simulink model "battery"  (R2024a)
settings: Solver=ode23t  StartTime=0.0  StopTime=10000.0  MaxStep=5e-2  RelTol=1e-3
undefined symbols (not defined in the file or in its folder): battery_builder_rtmsupport, gcbh
libraries: fl_lib x8, batt_lib x8, nesl_utility x6, Batteries_thermal_lib x6, SimscapeFluids_lib x1, simulink x1
(part 1 of 2)
settings Model: Creator=amtha  LastModifiedBy=amtha

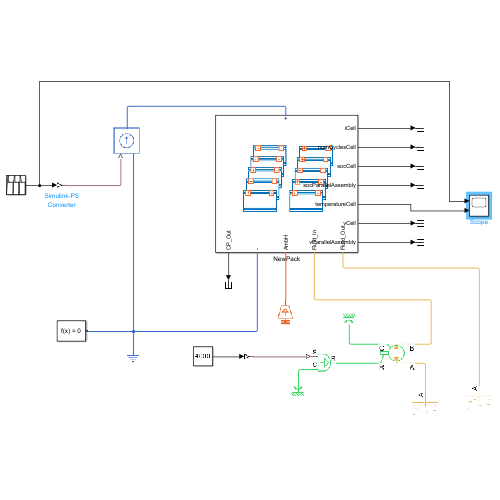
[thumbnail: Simulink's stored preview of the top-level diagram]
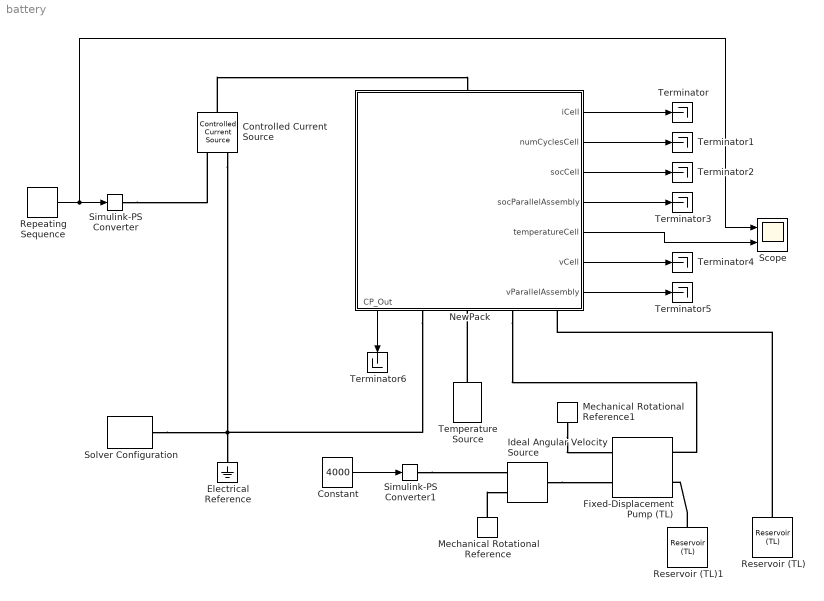
== system battery ==
  Constant : Constant  Value=4000
  Controlled Current Source : fl_lib/Electrical/Electrical Sources/Controlled Current Source
  Electrical Reference : fl_lib/Electrical/Electrical Elements/Electrical Reference
  Fixed-Displacement Pump (TL) : SimscapeFluids_lib/Thermal Liquid/Pumps & Motors/Fixed-Displacement Pump (TL)  loss_spec=fluids.thermal_liquid.pumps_motors.enum.LossSpec.Analytical  displacement=30 cm^3/rev  omega_nominal=4000 rpm  p_nominal=10 MPa  mu_nominal=0.9 cP  vol_eff_nominal=0.92  mech_eff_nominal=0.88  no_load_torque=0 N*m  p_diff_eff_TLU=[.1, 1, 2] MPa  omega_eff_TLU=[250, 500, 1000, 2000, 3000, 4000] rpm  vol_eff_TLU=[.816, .908, .954, .977, .981, .984; .325, .663, .831, .916, .925, .946; .137, .568, .78, .892, .893, .91]  mech_eff_TLU=[.996, .996, .996, .996, .996, .996; .988, .989, .989, .989, .989, .99; .981, .981, .982, .982, .983, .984]  p_diff_loss_TLU=[.1, 1, 2] MPa  omega_loss_TLU=[250, 500, 1000, 2000, 3000, 4000] rpm  vol_loss_TLU=1e-3 * [.023, .023, .023, .023, .0285, .032; .0844, .0842, .0845, .084, .1125, .108; .1079, .108, .11, .108, .1605, .18] m^3/s  mech_loss_TLU=[.002, .002, .002, .002, .002, .002; .0607, .0556, .0556, .0556, .0556, .0505; .1937, .1937, .1833, .1833, .1729, .1626] N*m  vol_eff_min=1e-3  vol_eff_max=1  mech_eff_min=1e-3  mech_eff_max=1  pressure_threshold=1e-3 MPa  omega_threshold=100 rpm  area=4.9087 cm^2  supplied_range_check=simscape.enum.assert.action.none  pump_mode_check=simscape.enum.assert.action.none
  Ideal Angular Velocity Source : fl_lib/Mechanical/Mechanical Sources/Ideal Angular Velocity Source
  Mechanical Rotational Reference : fl_lib/Mechanical/Rotational Elements/Mechanical Rotational Reference
  Mechanical Rotational Reference1 : fl_lib/Mechanical/Rotational Elements/Mechanical Rotational Reference
  NewPack : Subsystem  LoadFcn=battery_builder_rtmsupport('loadfcn',gcbh);
      settings: CopyFcn=battery_builder_rtmsupport('copyfcn',gcbh);  PreCopyFcn=battery_builder_rtmsupport('precopyfcn',gcbh);  PreDeleteFcn=battery_builder_rtmsupport('predeletefcn',gcbh);  PortSchema="{\"entries\":[{\"content\":{\"sides\":[{\"content\":{\"connectorIds\":[\"LConn1\"]},\"type\":\"ConnectorPlacement.EquallySpacedRectSide\",\"uuid\":\"1e77f675-d87b-42aa-aa84-96264be7bb8b\"},{\"content\":{\"connectorIds\":[\"Out1\",\"RConn1\",\"RConn2\",\"RConn3\",\"RConn4\"],\"side\":\"RIGHT\"},\"type\":\"ConnectorPlacement.EquallySpacedRectSide\",\"uuid\":\"6d3cd395-a28c-44d8-a256-e39544efc771\"},{\"content\":{\"side\":\"TOP\"},\"type\":\"ConnectorPlacement.EquallySpacedRectSide\",\"uuid\":\"362665c8-a493-42c4-a520-da428b1848bf\"},{\"content\":{\"connectorIds\":[\"Out2\",\"Out3\",\"Out4\",\"Out5\",\"Out6\",\"Out7\",\"Out8\"],\"side\":\"BOTTOM\"},\"type\":\"ConnectorPlacement.EquallySpacedRectSide\",\"uuid\":\"f34d4770-2d50-43cb-948c-fae9218760e2\"}]},\"type\":\"ConnectorPlacement.EquallySpacedConnector\",\"uuid\":\"a7a1b69c-e4ee-453d-b7ec-7a49ac1cf5a9\"}],\"packageUris\":[\"http://schema.mathworks.com/mf0/Connector/R2020b\"],\"version\":\"1.0\"}"
      mask Display: image('$imagefile')
  Repeating Sequence : simulink/Sources/Repeating Sequence  rep_seq_t=[0 500 1000 1500 2000 3000 3500 4000 5000 10000]  rep_seq_y=[-10 -10 0 0 5 5 0 0 0 0]
  Reservoir (TL) : fl_lib/Thermal Liquid/Elements/Reservoir (TL)  pressure_spec=foundation.enum.pressure_spec.atmospheric  reservoir_pressure=0.101325 MPa  reservoir_temperature=293.15 K  area=0.01 m^2
  Reservoir (TL)1 : fl_lib/Thermal Liquid/Elements/Reservoir (TL)  pressure_spec=foundation.enum.pressure_spec.atmospheric  reservoir_pressure=0.101325 MPa  reservoir_temperature=30 degC  area=0.01 m^2
  Scope : Scope  NumInputPorts=2
  Simulink-PS Converter : nesl_utility/Simulink-PS Converter  PhysicalDomain=network_engine_domain  SubClassName=ps_input  LeftPortType=input  RightPortType=output  PseudoPeriodic=off  Frequencies=[]  NoiseDistribution=none  NoiseParameters=[]  Unit=1  AffineConversion=off  FilteringAndDerivatives=provide  SimscapeFilterOrder=1  InputFilterTimeConstant=0.001  UdotUserProvided=0
  Simulink-PS Converter1 : nesl_utility/Simulink-PS Converter  PhysicalDomain=network_engine_domain  SubClassName=ps_input  LeftPortType=input  RightPortType=output  PseudoPeriodic=off  Frequencies=[]  NoiseDistribution=none  NoiseParameters=[]  Unit=1  AffineConversion=off  FilteringAndDerivatives=provide  SimscapeFilterOrder=1  InputFilterTimeConstant=0.001  UdotUserProvided=0
  Solver Configuration : nesl_utility/Solver Configuration  PhysicalDomain=network_engine_domain  SubClassName=solver  LeftPortType=input  RightPortType=generic  Tones=[]  Harmonics=[]  SimulateNoise=off  Profile=off  UseLocalSampling=off  EnableSwitchedLinearOptims=on  FrequencyDomain=off  UseCCode=off  RelTol=0.001  AbsTol=0.001  MinStep=1e-09  ToWorkspace=off  RevertToSquareIcSolve=off  NumHomotopyIterations=100  PhasorMode=off  PhasorModeNumHarmonics=1  ConsistencySolver=NEWTON_XTOL_AFTER_FTOL  IndexReductionMethod=DerivativeReplacement  DoDC=off  ResidualTolerance=1e-09  ConsistencyTolSource=GLOBAL  ConsistencyAbsTol=0.001  ConsistencyRelTol=0.001  ConsistencyTolFactor=0.001  UseLocalSolver=off  LocalSolverChoice=NE_BACKWARD_EULER_ADVANCER  ResolveIndetEquations=on  FunctionEvalNumThread=1  LocalSolverSampleTime=0.001  DoFixedCost=off  MaxNonlinIter=3  MaxModeIter=2  ComputeImpulses=off  ImpulseIterations=2  LinearAlgebra=auto  LinearAlgebraNumThread=0  EquationFormulation=NE_TIME_EF  DelaysMemoryBudget=1024  AutomaticFiltering=on  FilteringTimeConstant=0.001  PartitionStorageMethod=AS_NEEDED  PartitionMemoryBudget=1024  PartitionMethod=ROBUST  MultibodyUseLocalSolver=off  MultibodyLocalSolverChoice=ODE1  MultibodyLocalSolverSampleTime=0.001
  Temperature Source : fl_lib/Thermal/Thermal Sources/Temperature Source  temperature=293.15 K
  Terminator{,1..6} (7 alike) : Terminator
  wires:
  NewPack/2(iCell) -> Terminator/1
  NewPack/3(numCyclesCell) -> Terminator1/1
  NewPack/4(socCell) -> Terminator2/1
  NewPack/5(socParallelAssembly) -> Terminator3/1
  NewPack/7(vCell) -> Terminator4/1
  NewPack/8(vParallelAssembly) -> Terminator5/1
  NewPack/1(CP_Out) -> Terminator6/1
  Repeating Sequence/1 -> Scope/1, Simulink-PS Converter/1
  NewPack/6(temperatureCell) -> Scope/2
  Constant/1 -> Simulink-PS Converter1/1
  connections:
  Simulink-PS Converter/RConn1 -- Controlled Current Source/RConn1
  Controlled Current Source/RConn2 -- Solver Configuration/RConn1 -- NewPack/RConn1 -- Electrical Reference/LConn1
  Controlled Current Source/LConn1 -- NewPack/LConn1
  Simulink-PS Converter1/RConn1 -- Ideal Angular Velocity Source/RConn1
  Mechanical Rotational Reference/LConn1 -- Ideal Angular Velocity Source/RConn2
  Ideal Angular Velocity Source/LConn1 -- Fixed-Displacement Pump (TL)/RConn1
  Mechanical Rotational Reference1/LConn1 -- Fixed-Displacement Pump (TL)/RConn2
  NewPack/RConn3 -- Fixed-Displacement Pump (TL)/LConn2
  Reservoir (TL)/LConn1 -- NewPack/RConn4
  Reservoir (TL)1/LConn1 -- Fixed-Displacement Pump (TL)/LConn1
  Temperature Source/LConn1 -- NewPack/RConn2

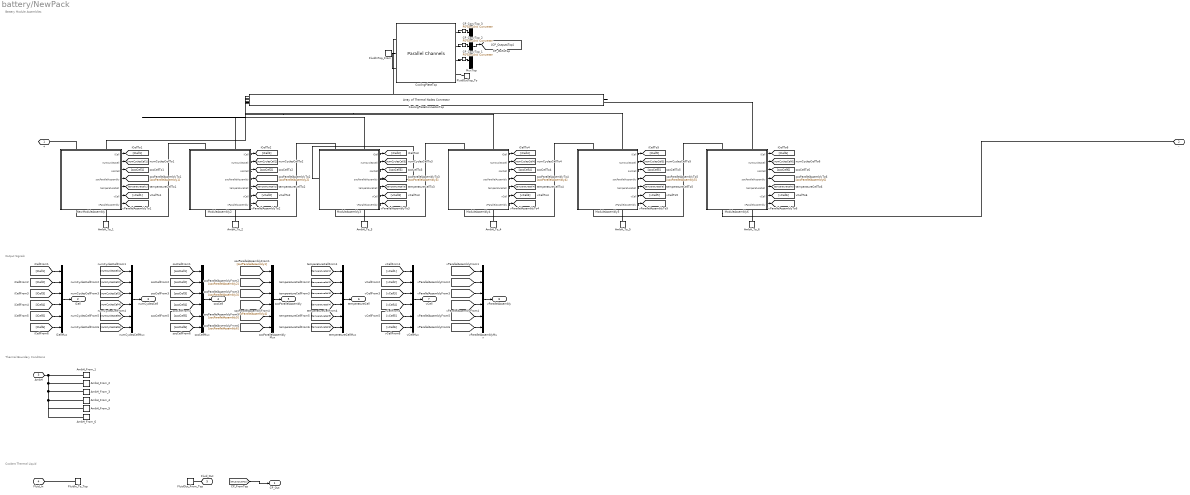
== system battery/NewPack ==
  note: Battery Module Assemblies
  note: Output Signals
  note: Thermal Boundary Conditions
  note: Coolant Thermal Liquid
  AmbH_From_1 : ConnectionLabel  Label=ambH_1
  AmbH_From_2 : ConnectionLabel  Label=ambH_2
  AmbH_From_3 : ConnectionLabel  Label=ambH_3
  AmbH_From_4 : ConnectionLabel  Label=ambH_4
  AmbH_From_5 : ConnectionLabel  Label=ambH_5
  AmbH_From_6 : ConnectionLabel  Label=ambH_6
  AmbH_To_1 : ConnectionLabel  Label=ambH_1
  AmbH_To_2 : ConnectionLabel  Label=ambH_2
  AmbH_To_3 : ConnectionLabel  Label=ambH_3
  AmbH_To_4 : ConnectionLabel  Label=ambH_4
  AmbH_To_5 : ConnectionLabel  Label=ambH_5
  AmbH_To_6 : ConnectionLabel  Label=ambH_6
  CP_ConvTop_1 : nesl_utility/PS-Simulink Converter  PhysicalDomain=network_engine_domain  SubClassName=ps_output  LeftPortType=input  RightPortType=output  PseudoPeriodic=off  Frequencies=[]  VectorFormat=inherit  Unit=inherit  AffineConversion=off
  CP_ConvTop_2 : nesl_utility/PS-Simulink Converter  PhysicalDomain=network_engine_domain  SubClassName=ps_output  LeftPortType=input  RightPortType=output  PseudoPeriodic=off  Frequencies=[]  VectorFormat=inherit  Unit=inherit  AffineConversion=off
  CP_ConvTop_3 : nesl_utility/PS-Simulink Converter  PhysicalDomain=network_engine_domain  SubClassName=ps_output  LeftPortType=input  RightPortType=output  PseudoPeriodic=off  Frequencies=[]  VectorFormat=inherit  Unit=inherit  AffineConversion=off
  CoolingPlateConnectorTop : batt_lib/Thermal/Array of Thermal Nodes Connector  numInputConnections=6  inNode1NumElements=1  inNode2NumElements=1  inNode3NumElements=1  inNode4NumElements=1  inNode5NumElements=1  inNode6NumElements=1  inNode7NumElements=1  inNode8NumElements=1  inNode9NumElements=1  inNode10NumElements=1  inNode11NumElements=1  inNode12NumElements=1  inNode13NumElements=1  inNode14NumElements=1  inNode15NumElements=1  inNode16NumElements=1  inNode17NumElements=1  inNode18NumElements=1  inNode19NumElements=1  inNode20NumElements=1  inNode21NumElements=1  inNode22NumElements=1  inNode23NumElements=1  inNode24NumElements=1  inNode25NumElements=1  inNode26NumElements=1  inNode27NumElements=1  inNode28NumElements=1  inNode29NumElements=1  inNode30NumElements=1  inNode31NumElements=1  inNode32NumElements=1  inNode33NumElements=1  inNode34NumElements=1  inNode35NumElements=1  inNode36NumElements=1  inNode37NumElements=1  inNode38NumElements=1  inNode39NumElements=1  inNode40NumElements=1  inNode41NumElements=1  inNode42NumElements=1  inNode43NumElements=1  inNode44NumElements=1  inNode45NumElements=1  inNode46NumElements=1  inNode47NumElements=1  inNode48NumElements=1  inNode49NumElements=1  inNode50NumElements=1
      settings: InternalSimscapePortConfiguration="{\"Bottom\":[{\"id\":\"outConn\",\"label\":\"outConn\",\"type\":\"foundation.thermal.thermal\"}],\"Left\":[],\"Right\":[],\"Top\":[{\"id\":\"inConn1\",\"label\":\"inConn1\",\"type\":\"foundation.thermal.thermal\"},{\"id\":\"inConn2\",\"label\":\"inConn2\",\"type\":\"foundation.thermal.thermal\"},{\"id\":\"inConn3\",\"label\":\"inConn3\",\"type\":\"foundation.thermal.thermal\"},{\"id\":\"inConn4\",\"label\":\"inConn4\",\"type\":\"foundation.thermal.thermal\"},{\"id\":\"inConn5\",\"label\":\"inConn5\",\"type\":\"foundation.thermal.thermal\"},{\"id\":\"inConn6\",\"label\":\"inConn6\",\"type\":\"foundation.thermal.thermal\"}]}"
  CoolingPlateTop : batt_lib/Thermal/Parallel Channels  plateConnectivity=simscape.battery.enum.thermal.coolingPlateConnectivity.singleSided  numBattThermalNodes1=6  dimensionThermalNodes1=[[0.0181 0.0181;0.0181 0.0181;0.0181 0.0181;0.0181 0.0181;0.0181 0.0181;0.0181 0.0181]]  locationThermalNodes1=[[0.00905 0.00905;0.02815 0.00905;0.04725 0.00905;0.06635 0.00905;0.08545 0.00905;0.10455 0.00905]]  numBattThermalNodes2=1  dimensionThermalNodes2=ones(1, 2)  locationThermalNodes2=ones(1, 2)  plateDimX=2  plateDimY=6  plateTh=2e-3 m  plateThCond=20 W/(K*m)  plateDen=2500 kg/m^3  plateCp=447 J/(K*kg)  plateTemp_ini=300 K  Re_lam=2000  Re_tur=4000  Nu_lam=3.66  length_add=1e-3 m  shape_factor=64  nChannels=4  selectChannelOrientation=simscape.battery.enum.thermal.coolingChannelsDirection.alongX  channelDia=0.92 m  distributorDia=0.92 m  roughnessPipe=1.5e-05 m
      settings: InternalSimscapePortConfiguration="{\"Bottom\":[],\"Left\":[{\"id\":\"fluid_in\",\"label\":\"fluid_in\",\"type\":\"foundation.thermal_liquid.thermal_liquid\"}],\"Right\":[{\"id\":\"fluid_out\",\"label\":\"fluid_out\",\"type\":\"foundation.thermal_liquid.thermal_liquid\"},{\"id\":\"plotPlateT\",\"label\":\"Tp\",\"type\":\"output\"},{\"id\":\"tempSensor\",\"label\":\"dT\",\"type\":\"output\"},{\"id\":\"presSensor\",\"label\":\"dP\",\"type\":\"output\"}],\"Top\":[{\"id\":\"Side1\",\"label\":\"Surf1\",\"type\":\"foundation.thermal.thermal\"}]}"
  FluidInTop_From : ConnectionLabel  Label=FluidIn_To_Top
  FluidIn_To_Top : ConnectionLabel  Label=FluidIn_To_Top
  FluidOutTop_To : ConnectionLabel  Label=FluidOut_From_Top
  FluidOut_From_Top : ConnectionLabel  Label=FluidOut_From_Top
  ModuleAssembly2 : Subsystem  LoadFcn=battery_builder_rtmsupport('loadfcn',gcbh);
      settings: CopyFcn=battery_builder_rtmsupport('copyfcn',gcbh);  PreCopyFcn=battery_builder_rtmsupport('precopyfcn',gcbh);  PreDeleteFcn=battery_builder_rtmsupport('predeletefcn',gcbh);  PortSchema="{\"entries\":[{\"content\":{\"sides\":[{\"content\":{\"connectorIds\":[\"LConn1\",\"LConn2\"]},\"type\":\"ConnectorPlacement.EquallySpacedRectSide\",\"uuid\":\"eec1a3b9-3cb1-4fa3-8fbd-a5fa5e4610c1\"},{\"content\":{\"connectorIds\":[\"RConn1\",\"RConn2\"],\"side\":\"RIGHT\"},\"type\":\"ConnectorPlacement.EquallySpacedRectSide\",\"uuid\":\"9ac1a2b7-e5b0-4055-8996-c7a8d7148ece\"},{\"content\":{\"side\":\"TOP\"},\"type\":\"ConnectorPlacement.EquallySpacedRectSide\",\"uuid\":\"c5219022-aec0-47d0-97c2-128c4c857f85\"},{\"content\":{\"connectorIds\":[\"Out1\",\"Out2\",\"Out3\",\"Out4\",\"Out5\",\"Out6\",\"Out7\"],\"side\":\"BOTTOM\"},\"type\":\"ConnectorPlacement.EquallySpacedRectSide\",\"uuid\":\"08f7c1a5-7ffe-4d76-b79a-02b9721237e6\"}]},\"type\":\"ConnectorPlacement.EquallySpacedConnector\",\"uuid\":\"b74244ab-6d11-4277-810b-3ebfddc08341\"}],\"packageUris\":[\"http://schema.mathworks.com/mf0/Connector/R2020b\"],\"version\":\"1.0\"}"
      mask Display: image('$imagefile')
  ModuleAssembly3 : Subsystem  LoadFcn=battery_builder_rtmsupport('loadfcn',gcbh);
      settings: CopyFcn=battery_builder_rtmsupport('copyfcn',gcbh);  PreCopyFcn=battery_builder_rtmsupport('precopyfcn',gcbh);  PreDeleteFcn=battery_builder_rtmsupport('predeletefcn',gcbh);  PortSchema="{\"entries\":[{\"content\":{\"sides\":[{\"content\":{\"connectorIds\":[\"LConn1\",\"LConn2\"]},\"type\":\"ConnectorPlacement.EquallySpacedRectSide\",\"uuid\":\"eec1a3b9-3cb1-4fa3-8fbd-a5fa5e4610c1\"},{\"content\":{\"connectorIds\":[\"RConn1\",\"RConn2\"],\"side\":\"RIGHT\"},\"type\":\"ConnectorPlacement.EquallySpacedRectSide\",\"uuid\":\"9ac1a2b7-e5b0-4055-8996-c7a8d7148ece\"},{\"content\":{\"side\":\"TOP\"},\"type\":\"ConnectorPlacement.EquallySpacedRectSide\",\"uuid\":\"c5219022-aec0-47d0-97c2-128c4c857f85\"},{\"content\":{\"connectorIds\":[\"Out1\",\"Out2\",\"Out3\",\"Out4\",\"Out5\",\"Out6\",\"Out7\"],\"side\":\"BOTTOM\"},\"type\":\"ConnectorPlacement.EquallySpacedRectSide\",\"uuid\":\"08f7c1a5-7ffe-4d76-b79a-02b9721237e6\"}]},\"type\":\"ConnectorPlacement.EquallySpacedConnector\",\"uuid\":\"b74244ab-6d11-4277-810b-3ebfddc08341\"}],\"packageUris\":[\"http://schema.mathworks.com/mf0/Connector/R2020b\"],\"version\":\"1.0\"}"
      mask Display: image('$imagefile')
  ModuleAssembly4 : Subsystem  LoadFcn=battery_builder_rtmsupport('loadfcn',gcbh);
      settings: CopyFcn=battery_builder_rtmsupport('copyfcn',gcbh);  PreCopyFcn=battery_builder_rtmsupport('precopyfcn',gcbh);  PreDeleteFcn=battery_builder_rtmsupport('predeletefcn',gcbh);  PortSchema="{\"entries\":[{\"content\":{\"sides\":[{\"content\":{\"connectorIds\":[\"LConn1\",\"LConn2\"]},\"type\":\"ConnectorPlacement.EquallySpacedRectSide\",\"uuid\":\"eec1a3b9-3cb1-4fa3-8fbd-a5fa5e4610c1\"},{\"content\":{\"connectorIds\":[\"RConn1\",\"RConn2\"],\"side\":\"RIGHT\"},\"type\":\"ConnectorPlacement.EquallySpacedRectSide\",\"uuid\":\"9ac1a2b7-e5b0-4055-8996-c7a8d7148ece\"},{\"content\":{\"side\":\"TOP\"},\"type\":\"ConnectorPlacement.EquallySpacedRectSide\",\"uuid\":\"c5219022-aec0-47d0-97c2-128c4c857f85\"},{\"content\":{\"connectorIds\":[\"Out1\",\"Out2\",\"Out3\",\"Out4\",\"Out5\",\"Out6\",\"Out7\"],\"side\":\"BOTTOM\"},\"type\":\"ConnectorPlacement.EquallySpacedRectSide\",\"uuid\":\"08f7c1a5-7ffe-4d76-b79a-02b9721237e6\"}]},\"type\":\"ConnectorPlacement.EquallySpacedConnector\",\"uuid\":\"b74244ab-6d11-4277-810b-3ebfddc08341\"}],\"packageUris\":[\"http://schema.mathworks.com/mf0/Connector/R2020b\"],\"version\":\"1.0\"}"
      mask Display: image('$imagefile')
  ModuleAssembly5 : Subsystem  LoadFcn=battery_builder_rtmsupport('loadfcn',gcbh);
      settings: CopyFcn=battery_builder_rtmsupport('copyfcn',gcbh);  PreCopyFcn=battery_builder_rtmsupport('precopyfcn',gcbh);  PreDeleteFcn=battery_builder_rtmsupport('predeletefcn',gcbh);  PortSchema="{\"entries\":[{\"content\":{\"sides\":[{\"content\":{\"connectorIds\":[\"LConn1\",\"LConn2\"]},\"type\":\"ConnectorPlacement.EquallySpacedRectSide\",\"uuid\":\"eec1a3b9-3cb1-4fa3-8fbd-a5fa5e4610c1\"},{\"content\":{\"connectorIds\":[\"RConn1\",\"RConn2\"],\"side\":\"RIGHT\"},\"type\":\"ConnectorPlacement.EquallySpacedRectSide\",\"uuid\":\"9ac1a2b7-e5b0-4055-8996-c7a8d7148ece\"},{\"content\":{\"side\":\"TOP\"},\"type\":\"ConnectorPlacement.EquallySpacedRectSide\",\"uuid\":\"c5219022-aec0-47d0-97c2-128c4c857f85\"},{\"content\":{\"connectorIds\":[\"Out1\",\"Out2\",\"Out3\",\"Out4\",\"Out5\",\"Out6\",\"Out7\"],\"side\":\"BOTTOM\"},\"type\":\"ConnectorPlacement.EquallySpacedRectSide\",\"uuid\":\"08f7c1a5-7ffe-4d76-b79a-02b9721237e6\"}]},\"type\":\"ConnectorPlacement.EquallySpacedConnector\",\"uuid\":\"b74244ab-6d11-4277-810b-3ebfddc08341\"}],\"packageUris\":[\"http://schema.mathworks.com/mf0/Connector/R2020b\"],\"version\":\"1.0\"}"
      mask Display: image('$imagefile')
  ModuleAssembly6 : Subsystem  LoadFcn=battery_builder_rtmsupport('loadfcn',gcbh);
      settings: CopyFcn=battery_builder_rtmsupport('copyfcn',gcbh);  PreCopyFcn=battery_builder_rtmsupport('precopyfcn',gcbh);  PreDeleteFcn=battery_builder_rtmsupport('predeletefcn',gcbh);  PortSchema="{\"entries\":[{\"content\":{\"sides\":[{\"content\":{\"connectorIds\":[\"LConn1\",\"LConn2\"]},\"type\":\"ConnectorPlacement.EquallySpacedRectSide\",\"uuid\":\"eec1a3b9-3cb1-4fa3-8fbd-a5fa5e4610c1\"},{\"content\":{\"connectorIds\":[\"RConn1\",\"RConn2\"],\"side\":\"RIGHT\"},\"type\":\"ConnectorPlacement.EquallySpacedRectSide\",\"uuid\":\"9ac1a2b7-e5b0-4055-8996-c7a8d7148ece\"},{\"content\":{\"side\":\"TOP\"},\"type\":\"ConnectorPlacement.EquallySpacedRectSide\",\"uuid\":\"c5219022-aec0-47d0-97c2-128c4c857f85\"},{\"content\":{\"connectorIds\":[\"Out1\",\"Out2\",\"Out3\",\"Out4\",\"Out5\",\"Out6\",\"Out7\"],\"side\":\"BOTTOM\"},\"type\":\"ConnectorPlacement.EquallySpacedRectSide\",\"uuid\":\"08f7c1a5-7ffe-4d76-b79a-02b9721237e6\"}]},\"type\":\"ConnectorPlacement.EquallySpacedConnector\",\"uuid\":\"b74244ab-6d11-4277-810b-3ebfddc08341\"}],\"packageUris\":[\"http://schema.mathworks.com/mf0/Connector/R2020b\"],\"version\":\"1.0\"}"
      mask Display: image('$imagefile')
  MuxTop : Mux  Inputs=3
  NewModuleAssembly : Subsystem  LoadFcn=battery_builder_rtmsupport('loadfcn',gcbh);
      settings: CopyFcn=battery_builder_rtmsupport('copyfcn',gcbh);  PreCopyFcn=battery_builder_rtmsupport('precopyfcn',gcbh);  PreDeleteFcn=battery_builder_rtmsupport('predeletefcn',gcbh);  PortSchema="{\"entries\":[{\"content\":{\"sides\":[{\"content\":{\"connectorIds\":[\"LConn1\",\"LConn2\"]},\"type\":\"ConnectorPlacement.EquallySpacedRectSide\",\"uuid\":\"eec1a3b9-3cb1-4fa3-8fbd-a5fa5e4610c1\"},{\"content\":{\"connectorIds\":[\"RConn1\",\"RConn2\"],\"side\":\"RIGHT\"},\"type\":\"ConnectorPlacement.EquallySpacedRectSide\",\"uuid\":\"9ac1a2b7-e5b0-4055-8996-c7a8d7148ece\"},{\"content\":{\"side\":\"TOP\"},\"type\":\"ConnectorPlacement.EquallySpacedRectSide\",\"uuid\":\"c5219022-aec0-47d0-97c2-128c4c857f85\"},{\"content\":{\"connectorIds\":[\"Out1\",\"Out2\",\"Out3\",\"Out4\",\"Out5\",\"Out6\",\"Out7\"],\"side\":\"BOTTOM\"},\"type\":\"ConnectorPlacement.EquallySpacedRectSide\",\"uuid\":\"08f7c1a5-7ffe-4d76-b79a-02b9721237e6\"}]},\"type\":\"ConnectorPlacement.EquallySpacedConnector\",\"uuid\":\"b74244ab-6d11-4277-810b-3ebfddc08341\"}],\"packageUris\":[\"http://schema.mathworks.com/mf0/Connector/R2020b\"],\"version\":\"1.0\"}"
      mask Display: image('$imagefile')
  iCellMux : Mux  Inputs=6
  numCyclesCellMux : Mux  Inputs=6
  socCellMux : Mux  Inputs=6
  socParallelAssemblyMux : Mux  Inputs=6
  temperatureCellMux : Mux  Inputs=6
  vCellMux : Mux  Inputs=6
  vParallelAssemblyMux : Mux  Inputs=6
  + : PMIOPort  Side=Left
  - : PMIOPort  Port=2  Side=Right
  AmbH : PMIOPort  Port=3  Side=Right  ConnectionType=Connection: foundation.thermal.thermal
  Fluid_In : PMIOPort  Port=4  Side=Right  ConnectionType=Connection: foundation.thermal_liquid.thermal_liquid
  Fluid_Out : PMIOPort  Port=5  Side=Right  ConnectionType=Connection: foundation.thermal_liquid.thermal_liquid
  CP_Out : Outport
  iCell : Outport  Port=2
  numCyclesCell : Outport  Port=3
  socCell : Outport  Port=4
  socParallelAssembly : Outport  Port=5
  temperatureCell : Outport  Port=6
  vCell : Outport  Port=7
  vParallelAssembly : Outport  Port=8
  wires:
  NewModuleAssembly/1(iCell) -> [iCell1]
  iCellMux/1 -> iCell/1
  [iCell1] -> iCellMux/1
  NewModuleAssembly/2(numCyclesCell) -> [numCyclesCell1]
  numCyclesCellMux/1 -> numCyclesCell/1
  [numCyclesCell1] -> numCyclesCellMux/1
  NewModuleAssembly/3(socCell) -> [socCell1]
  socCellMux/1 -> socCell/1
  [socCell1] -> socCellMux/1
  NewModuleAssembly/4(socParallelAssembly) -> [socParallelAssembly1]
  socParallelAssemblyMux/1 -> socParallelAssembly/1
  [socParallelAssembly1] -> socParallelAssemblyMux/1
  NewModuleAssembly/5(temperatureCell) -> [temperatureCell1]
  temperatureCellMux/1 -> temperatureCell/1
  [temperatureCell1] -> temperatureCellMux/1
  NewModuleAssembly/6(vCell) -> [vCell1]
  vCellMux/1 -> vCell/1
  [vCell1] -> vCellMux/1
  NewModuleAssembly/7(vParallelAssembly) -> [vParallelAssembly1]
  vParallelAssemblyMux/1 -> vParallelAssembly/1
  [vParallelAssembly1] -> vParallelAssemblyMux/1
  ModuleAssembly2/1(iCell) -> [iCell2]
  [iCell2] -> iCellMux/2
  ModuleAssembly2/2(numCyclesCell) -> [numCyclesCell2]
  [numCyclesCell2] -> numCyclesCellMux/2
  ModuleAssembly2/3(socCell) -> [socCell2]
  [socCell2] -> socCellMux/2
  ModuleAssembly2/4(socParallelAssembly) -> [socParallelAssembly2]
  [socParallelAssembly2] -> socParallelAssemblyMux/2
  ModuleAssembly2/5(temperatureCell) -> [temperatureCell2]
  [temperatureCell2] -> temperatureCellMux/2
  ModuleAssembly2/6(vCell) -> [vCell2]
  [vCell2] -> vCellMux/2
  ModuleAssembly2/7(vParallelAssembly) -> [vParallelAssembly2]
  [vParallelAssembly2] -> vParallelAssemblyMux/2
  ModuleAssembly3/1(iCell) -> [iCell3]
  [iCell3] -> iCellMux/3
  ModuleAssembly3/2(numCyclesCell) -> [numCyclesCell3]
  [numCyclesCell3] -> numCyclesCellMux/3
  ModuleAssembly3/3(socCell) -> [socCell3]
  [socCell3] -> socCellMux/3
  ModuleAssembly3/4(socParallelAssembly) -> [socParallelAssembly3]
  [socParallelAssembly3] -> socParallelAssemblyMux/3
  ModuleAssembly3/5(temperatureCell) -> [temperatureCell3]
  [temperatureCell3] -> temperatureCellMux/3
  ModuleAssembly3/6(vCell) -> [vCell3]
  [vCell3] -> vCellMux/3
  ModuleAssembly3/7(vParallelAssembly) -> [vParallelAssembly3]
  [vParallelAssembly3] -> vParallelAssemblyMux/3
  ModuleAssembly4/1(iCell) -> [iCell4]
  [iCell4] -> iCellMux/4
  ModuleAssembly4/2(numCyclesCell) -> [numCyclesCell4]
  [numCyclesCell4] -> numCyclesCellMux/4
  ModuleAssembly4/3(socCell) -> [socCell4]
  [socCell4] -> socCellMux/4
  ModuleAssembly4/4(socParallelAssembly) -> [socParallelAssembly4]
  [socParallelAssembly4] -> socParallelAssemblyMux/4
  ModuleAssembly4/5(temperatureCell) -> [temperatureCell4]
  [temperatureCell4] -> temperatureCellMux/4
  ModuleAssembly4/6(vCell) -> [vCell4]
  [vCell4] -> vCellMux/4
  ModuleAssembly4/7(vParallelAssembly) -> [vParallelAssembly4]
  [vParallelAssembly4] -> vParallelAssemblyMux/4
  ModuleAssembly5/1(iCell) -> [iCell5]
  [iCell5] -> iCellMux/5
  ModuleAssembly5/2(numCyclesCell) -> [numCyclesCell5]
  [numCyclesCell5] -> numCyclesCellMux/5
  ModuleAssembly5/3(socCell) -> [socCell5]
  [socCell5] -> socCellMux/5
  ModuleAssembly5/4(socParallelAssembly) -> [socParallelAssembly5]
  [socParallelAssembly5] -> socParallelAssemblyMux/5
  ModuleAssembly5/5(temperatureCell) -> [temperatureCell5]
  [temperatureCell5] -> temperatureCellMux/5
  ModuleAssembly5/6(vCell) -> [vCell5]
  [vCell5] -> vCellMux/5
  ModuleAssembly5/7(vParallelAssembly) -> [vParallelAssembly5]
  [vParallelAssembly5] -> vParallelAssemblyMux/5
  ModuleAssembly6/1(iCell) -> [iCell6]
  [iCell6] -> iCellMux/6
  ModuleAssembly6/2(numCyclesCell) -> [numCyclesCell6]
  [numCyclesCell6] -> numCyclesCellMux/6
  ModuleAssembly6/3(socCell) -> [socCell6]
  [socCell6] -> socCellMux/6
  ModuleAssembly6/4(socParallelAssembly) -> [socParallelAssembly6]
  [socParallelAssembly6] -> socParallelAssemblyMux/6
  ModuleAssembly6/5(temperatureCell) -> [temperatureCell6]
  [temperatureCell6] -> temperatureCellMux/6
  ModuleAssembly6/6(vCell) -> [vCell6]
  [vCell6] -> vCellMux/6
  ModuleAssembly6/7(vParallelAssembly) -> [vParallelAssembly6]
  [vParallelAssembly6] -> vParallelAssemblyMux/6
  CP_ConvTop_1/1 -> MuxTop/3
  CP_ConvTop_2/1 -> MuxTop/2
  CP_ConvTop_3/1 -> MuxTop/1
  MuxTop/1 -> [CP_OutputsTop]
  [CP_OutputsTop] -> CP_Out/1
  connections:
  ModuleAssembly2/LConn1 -- NewModuleAssembly/RConn1
  ModuleAssembly3/LConn1 -- ModuleAssembly2/RConn1
  ModuleAssembly4/LConn1 -- ModuleAssembly3/RConn1
  ModuleAssembly5/LConn1 -- ModuleAssembly4/RConn1
  ModuleAssembly6/LConn1 -- ModuleAssembly5/RConn1
  NewModuleAssembly/LConn1 -- +/RConn1
  ModuleAssembly6/RConn1 -- -/RConn1
  AmbH_To_1/LConn1 -- NewModuleAssembly/RConn2
  AmbH_From_1/LConn1 -- AmbH_From_6/LConn1 -- AmbH_From_5/LConn1 -- AmbH_From_4/LConn1 -- AmbH_From_3/LConn1 -- AmbH_From_2/LConn1 -- AmbH/RConn1
  AmbH_To_2/LConn1 -- ModuleAssembly2/RConn2
  AmbH_To_3/LConn1 -- ModuleAssembly3/RConn2
  AmbH_To_4/LConn1 -- ModuleAssembly4/RConn2
  AmbH_To_5/LConn1 -- ModuleAssembly5/RConn2
  AmbH_To_6/LConn1 -- ModuleAssembly6/RConn2
  CoolingPlateConnectorTop/LConn1 -- NewModuleAssembly/LConn2
  CoolingPlateConnectorTop/LConn2 -- ModuleAssembly2/LConn2
  CoolingPlateConnectorTop/LConn3 -- ModuleAssembly3/LConn2
  CoolingPlateConnectorTop/LConn4 -- ModuleAssembly4/LConn2
  CoolingPlateConnectorTop/LConn5 -- ModuleAssembly5/LConn2
  CoolingPlateConnectorTop/LConn6 -- ModuleAssembly6/LConn2
  CoolingPlateConnectorTop/RConn1 -- CoolingPlateTop/LConn2
  FluidIn_To_Top/LConn1 -- Fluid_In/RConn1
  Fluid_Out/RConn1 -- FluidOut_From_Top/LConn1
  FluidInTop_From/LConn1 -- CoolingPlateTop/LConn1
  CoolingPlateTop/RConn1 -- FluidOutTop_To/LConn1
  CoolingPlateTop/RConn2 -- CP_ConvTop_1/LConn1
  CoolingPlateTop/RConn3 -- CP_ConvTop_2/LConn1
  CoolingPlateTop/RConn4 -- CP_ConvTop_3/LConn1

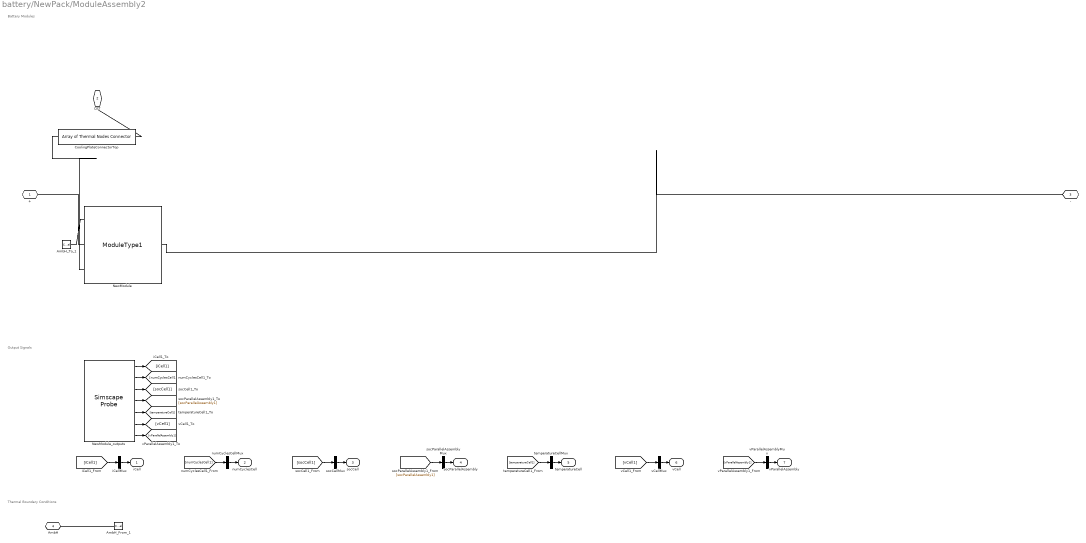
== system battery/NewPack/ModuleAssembly2 ==
  note: Thermal Boundary Conditions
  note: Output Signals
  note: Battery Modules
  AmbH_From_1 : ConnectionLabel  Label=ambH_1
  AmbH_To_1 : ConnectionLabel  Label=ambH_1
  CoolingPlateConnectorTop : batt_lib/Thermal/Array of Thermal Nodes Connector  numInputConnections=1  inNode1NumElements=1  inNode2NumElements=1  inNode3NumElements=1  inNode4NumElements=1  inNode5NumElements=1  inNode6NumElements=1  inNode7NumElements=1  inNode8NumElements=1  inNode9NumElements=1  inNode10NumElements=1  inNode11NumElements=1  inNode12NumElements=1  inNode13NumElements=1  inNode14NumElements=1  inNode15NumElements=1  inNode16NumElements=1  inNode17NumElements=1  inNode18NumElements=1  inNode19NumElements=1  inNode20NumElements=1  inNode21NumElements=1  inNode22NumElements=1  inNode23NumElements=1  inNode24NumElements=1  inNode25NumElements=1  inNode26NumElements=1  inNode27NumElements=1  inNode28NumElements=1  inNode29NumElements=1  inNode30NumElements=1  inNode31NumElements=1  inNode32NumElements=1  inNode33NumElements=1  inNode34NumElements=1  inNode35NumElements=1  inNode36NumElements=1  inNode37NumElements=1  inNode38NumElements=1  inNode39NumElements=1  inNode40NumElements=1  inNode41NumElements=1  inNode42NumElements=1  inNode43NumElements=1  inNode44NumElements=1  inNode45NumElements=1  inNode46NumElements=1  inNode47NumElements=1  inNode48NumElements=1  inNode49NumElements=1  inNode50NumElements=1
      settings: InternalSimscapePortConfiguration="{\"Bottom\":[{\"id\":\"outConn\",\"label\":\"outConn\",\"type\":\"foundation.thermal.thermal\"}],\"Left\":[],\"Right\":[],\"Top\":[{\"id\":\"inConn1\",\"label\":\"inConn1\",\"type\":\"foundation.thermal.thermal\"}]}"
  NewModule : Batteries_thermal_lib/Modules/ModuleType1  SOC_vecCell=[0, .1, .25, .5, .75, .9, 1]  T_vecCell=[278, 293, 313] K  V0_matCell=[3.49, 3.5, 3.51; 3.55, 3.57, 3.56; 3.62, 3.63, 3.64; 3.71, 3.71, 3.72; 3.91, 3.93, 3.94; 4.07, 4.08, 4.08; 4.19, 4.19, 4.19] V  V_rangeCell=[0, inf] V  R0_matCell=[.0117, .0085, .009; .011, .0085, .009; .0114, .0087, .0092; .0107, .0082, .0088; .0107, .0083, .0091; .0113, .0085, .0089; .0116, .0085, .0089] Ohm  AHCell=27 A*hr  extrapolation_optionCell=simscape.enum.extrapolation.nearest  thermal_massCell=100 J/K  CoolantResistance=1.2 K/W  AmbientResistance=25 K/W  P=1  S=1  iCell_specify=off  iCell_priority=None  iCell=0 A  iCell_nominal_specify=off  iCell_nominal_value=1  iCell_nominal_unit=A  vCell_specify=off  vCell_priority=None  vCell=0 V  vCell_nominal_specify=off  vCell_nominal_value=1  vCell_nominal_unit=V  socCell_specify=off  socCell_priority=High  socCell=1  socCell_nominal_specify=off  socCell_nominal_value=1  socCell_nominal_unit=1  numCyclesCell_specify=off  numCyclesCell_priority=High  numCyclesCell=0  numCyclesCell_nominal_specify=off  numCyclesCell_nominal_value=1  numCyclesCell_nominal_unit=1  temperatureCell_specify=off  temperatureCell_priority=High  temperatureCell=298.15 K  temperatureCell_nominal_specify=off  temperatureCell_nominal_value=1  temperatureCell_nominal_unit=K  vParallelAssembly_specify=off  vParallelAssembly_priority=None  vParallelAssembly=0 V  vParallelAssembly_nominal_specify=off  vParallelAssembly_nominal_value=1  vParallelAssembly_nominal_unit=V  socParallelAssembly_specify=off  socParallelAssembly_priority=None  socParallelAssembly=1  socParallelAssembly_nominal_specify=off  socParallelAssembly_nominal_value=1  socParallelAssembly_nominal_unit=1
      settings: InternalSimscapePortConfiguration="{\"Bottom\":[{\"id\":\"n\",\"label\":\"-\",\"type\":\"foundation.electrical.electrical\"}],\"Left\":[{\"id\":\"AmbH\",\"label\":\"AmbH\",\"type\":\"foundation.thermal.thermal\"}],\"Right\":[],\"Top\":[{\"id\":\"p\",\"label\":\"+\",\"type\":\"foundation.electrical.electrical\"},{\"id\":\"TopExtClnt\",\"label\":\"CPT\",\"type\":\"foundation.thermal.thermal\"}]}"
  NewModule_outputs : SimscapeProbe  BoundBlock=29  Variables={iCell, numCyclesCell, socCell, socParallelAssembly, temperatureCell, vCell, vParallelAssembly}
  iCellMux : Mux  Inputs=1
  numCyclesCellMux : Mux  Inputs=1
  socCellMux : Mux  Inputs=1
  socParallelAssemblyMux : Mux  Inputs=1
  temperatureCellMux : Mux  Inputs=1
  vCellMux : Mux  Inputs=1
  vParallelAssemblyMux : Mux  Inputs=1
  + : PMIOPort  Side=Left
  CPT : PMIOPort  Port=2  Side=Left  ConnectionType=Connection: foundation.thermal.thermal
  - : PMIOPort  Port=3  Side=Right
  AmbH : PMIOPort  Port=4  Side=Right  ConnectionType=Connection: foundation.thermal.thermal
  iCell : Outport
  numCyclesCell : Outport  Port=2
  socCell : Outport  Port=3
  socParallelAssembly : Outport  Port=4
  temperatureCell : Outport  Port=5
  vCell : Outport  Port=6
  vParallelAssembly : Outport  Port=7
  wires:
  [vParallelAssembly1] -> vParallelAssemblyMux/1
  vParallelAssemblyMux/1 -> vParallelAssembly/1
  NewModule_outputs/7 -> [vParallelAssembly1]
  [vCell1] -> vCellMux/1
  vCellMux/1 -> vCell/1
  NewModule_outputs/6 -> [vCell1]
  [temperatureCell1] -> temperatureCellMux/1
  temperatureCellMux/1 -> temperatureCell/1
  NewModule_outputs/5 -> [temperatureCell1]
  [socParallelAssembly1] -> socParallelAssemblyMux/1
  socParallelAssemblyMux/1 -> socParallelAssembly/1
  NewModule_outputs/4 -> [socParallelAssembly1]
  [socCell1] -> socCellMux/1
  socCellMux/1 -> socCell/1
  NewModule_outputs/3 -> [socCell1]
  [numCyclesCell1] -> numCyclesCellMux/1
  numCyclesCellMux/1 -> numCyclesCell/1
  NewModule_outputs/2 -> [numCyclesCell1]
  [iCell1] -> iCellMux/1
  iCellMux/1 -> iCell/1
  NewModule_outputs/1 -> [iCell1]
  connections:
  CoolingPlateConnectorTop/RConn1 -- CPT/RConn1
  CoolingPlateConnectorTop/LConn1 -- NewModule/LConn3
  AmbH_From_1/LConn1 -- AmbH/RConn1
  AmbH_To_1/LConn1 -- NewModule/LConn1
  NewModule/RConn1 -- -/RConn1
  NewModule/LConn2 -- +/RConn1

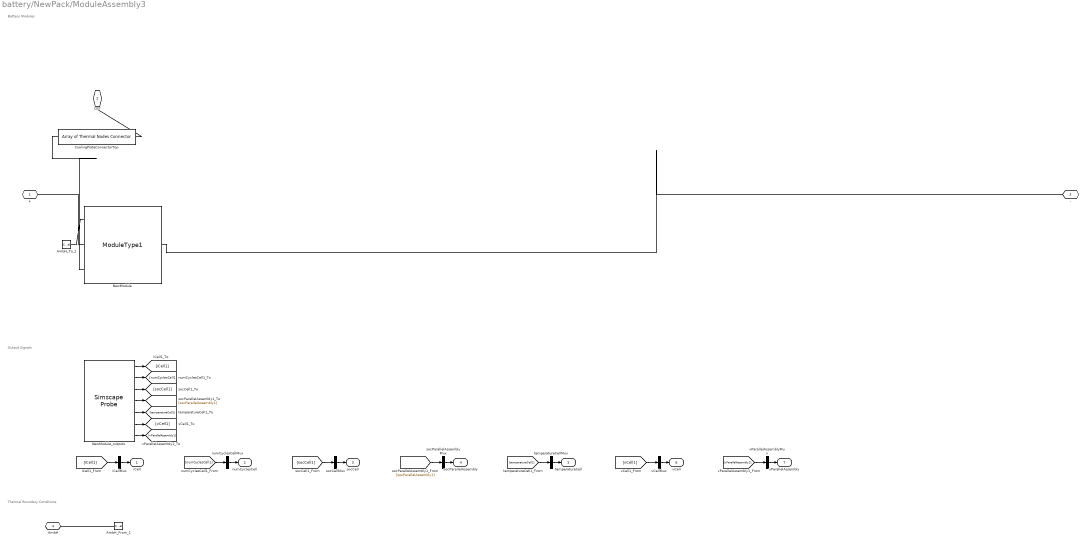
== system battery/NewPack/ModuleAssembly3 ==
  note: Thermal Boundary Conditions
  note: Output Signals
  note: Battery Modules
  AmbH_From_1 : ConnectionLabel  Label=ambH_1
  AmbH_To_1 : ConnectionLabel  Label=ambH_1
  CoolingPlateConnectorTop : batt_lib/Thermal/Array of Thermal Nodes Connector  numInputConnections=1  inNode1NumElements=1  inNode2NumElements=1  inNode3NumElements=1  inNode4NumElements=1  inNode5NumElements=1  inNode6NumElements=1  inNode7NumElements=1  inNode8NumElements=1  inNode9NumElements=1  inNode10NumElements=1  inNode11NumElements=1  inNode12NumElements=1  inNode13NumElements=1  inNode14NumElements=1  inNode15NumElements=1  inNode16NumElements=1  inNode17NumElements=1  inNode18NumElements=1  inNode19NumElements=1  inNode20NumElements=1  inNode21NumElements=1  inNode22NumElements=1  inNode23NumElements=1  inNode24NumElements=1  inNode25NumElements=1  inNode26NumElements=1  inNode27NumElements=1  inNode28NumElements=1  inNode29NumElements=1  inNode30NumElements=1  inNode31NumElements=1  inNode32NumElements=1  inNode33NumElements=1  inNode34NumElements=1  inNode35NumElements=1  inNode36NumElements=1  inNode37NumElements=1  inNode38NumElements=1  inNode39NumElements=1  inNode40NumElements=1  inNode41NumElements=1  inNode42NumElements=1  inNode43NumElements=1  inNode44NumElements=1  inNode45NumElements=1  inNode46NumElements=1  inNode47NumElements=1  inNode48NumElements=1  inNode49NumElements=1  inNode50NumElements=1
      settings: InternalSimscapePortConfiguration="{\"Bottom\":[{\"id\":\"outConn\",\"label\":\"outConn\",\"type\":\"foundation.thermal.thermal\"}],\"Left\":[],\"Right\":[],\"Top\":[{\"id\":\"inConn1\",\"label\":\"inConn1\",\"type\":\"foundation.thermal.thermal\"}]}"
  NewModule : Batteries_thermal_lib/Modules/ModuleType1  SOC_vecCell=[0, .1, .25, .5, .75, .9, 1]  T_vecCell=[278, 293, 313] K  V0_matCell=[3.49, 3.5, 3.51; 3.55, 3.57, 3.56; 3.62, 3.63, 3.64; 3.71, 3.71, 3.72; 3.91, 3.93, 3.94; 4.07, 4.08, 4.08; 4.19, 4.19, 4.19] V  V_rangeCell=[0, inf] V  R0_matCell=[.0117, .0085, .009; .011, .0085, .009; .0114, .0087, .0092; .0107, .0082, .0088; .0107, .0083, .0091; .0113, .0085, .0089; .0116, .0085, .0089] Ohm  AHCell=27 A*hr  extrapolation_optionCell=simscape.enum.extrapolation.nearest  thermal_massCell=100 J/K  CoolantResistance=1.2 K/W  AmbientResistance=25 K/W  P=1  S=1  iCell_specify=off  iCell_priority=None  iCell=0 A  iCell_nominal_specify=off  iCell_nominal_value=1  iCell_nominal_unit=A  vCell_specify=off  vCell_priority=None  vCell=0 V  vCell_nominal_specify=off  vCell_nominal_value=1  vCell_nominal_unit=V  socCell_specify=off  socCell_priority=High  socCell=1  socCell_nominal_specify=off  socCell_nominal_value=1  socCell_nominal_unit=1  numCyclesCell_specify=off  numCyclesCell_priority=High  numCyclesCell=0  numCyclesCell_nominal_specify=off  numCyclesCell_nominal_value=1  numCyclesCell_nominal_unit=1  temperatureCell_specify=off  temperatureCell_priority=High  temperatureCell=298.15 K  temperatureCell_nominal_specify=off  temperatureCell_nominal_value=1  temperatureCell_nominal_unit=K  vParallelAssembly_specify=off  vParallelAssembly_priority=None  vParallelAssembly=0 V  vParallelAssembly_nominal_specify=off  vParallelAssembly_nominal_value=1  vParallelAssembly_nominal_unit=V  socParallelAssembly_specify=off  socParallelAssembly_priority=None  socParallelAssembly=1  socParallelAssembly_nominal_specify=off  socParallelAssembly_nominal_value=1  socParallelAssembly_nominal_unit=1
      settings: InternalSimscapePortConfiguration="{\"Bottom\":[{\"id\":\"n\",\"label\":\"-\",\"type\":\"foundation.electrical.electrical\"}],\"Left\":[{\"id\":\"AmbH\",\"label\":\"AmbH\",\"type\":\"foundation.thermal.thermal\"}],\"Right\":[],\"Top\":[{\"id\":\"p\",\"label\":\"+\",\"type\":\"foundation.electrical.electrical\"},{\"id\":\"TopExtClnt\",\"label\":\"CPT\",\"type\":\"foundation.thermal.thermal\"}]}"
  NewModule_outputs : SimscapeProbe  BoundBlock=70  Variables={iCell, numCyclesCell, socCell, socParallelAssembly, temperatureCell, vCell, vParallelAssembly}
  iCellMux : Mux  Inputs=1
  numCyclesCellMux : Mux  Inputs=1
  socCellMux : Mux  Inputs=1
  socParallelAssemblyMux : Mux  Inputs=1
  temperatureCellMux : Mux  Inputs=1
  vCellMux : Mux  Inputs=1
  vParallelAssemblyMux : Mux  Inputs=1
  + : PMIOPort  Side=Left
  CPT : PMIOPort  Port=2  Side=Left  ConnectionType=Connection: foundation.thermal.thermal
  - : PMIOPort  Port=3  Side=Right
  AmbH : PMIOPort  Port=4  Side=Right  ConnectionType=Connection: foundation.thermal.thermal
  iCell : Outport
  numCyclesCell : Outport  Port=2
  socCell : Outport  Port=3
  socParallelAssembly : Outport  Port=4
  temperatureCell : Outport  Port=5
  vCell : Outport  Port=6
  vParallelAssembly : Outport  Port=7
  wires:
  [vParallelAssembly1] -> vParallelAssemblyMux/1
  vParallelAssemblyMux/1 -> vParallelAssembly/1
  NewModule_outputs/7 -> [vParallelAssembly1]
  [vCell1] -> vCellMux/1
  vCellMux/1 -> vCell/1
  NewModule_outputs/6 -> [vCell1]
  [temperatureCell1] -> temperatureCellMux/1
  temperatureCellMux/1 -> temperatureCell/1
  NewModule_outputs/5 -> [temperatureCell1]
  [socParallelAssembly1] -> socParallelAssemblyMux/1
  socParallelAssemblyMux/1 -> socParallelAssembly/1
  NewModule_outputs/4 -> [socParallelAssembly1]
  [socCell1] -> socCellMux/1
  socCellMux/1 -> socCell/1
  NewModule_outputs/3 -> [socCell1]
  [numCyclesCell1] -> numCyclesCellMux/1
  numCyclesCellMux/1 -> numCyclesCell/1
  NewModule_outputs/2 -> [numCyclesCell1]
  [iCell1] -> iCellMux/1
  iCellMux/1 -> iCell/1
  NewModule_outputs/1 -> [iCell1]
  connections:
  CoolingPlateConnectorTop/RConn1 -- CPT/RConn1
  CoolingPlateConnectorTop/LConn1 -- NewModule/LConn3
  AmbH_From_1/LConn1 -- AmbH/RConn1
  AmbH_To_1/LConn1 -- NewModule/LConn1
  NewModule/RConn1 -- -/RConn1
  NewModule/LConn2 -- +/RConn1

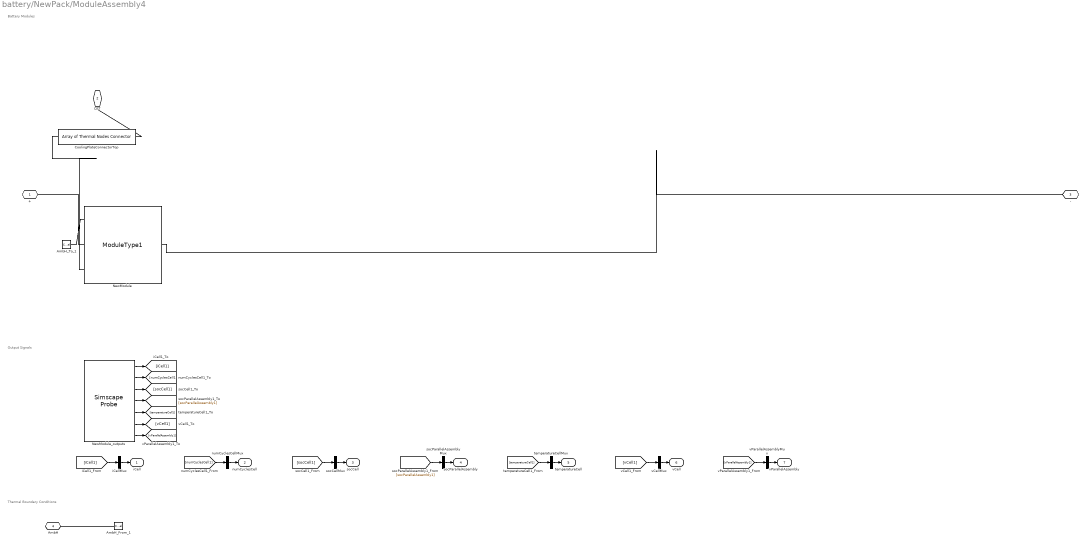
== system battery/NewPack/ModuleAssembly4 ==
  note: Thermal Boundary Conditions
  note: Output Signals
  note: Battery Modules
  AmbH_From_1 : ConnectionLabel  Label=ambH_1
  AmbH_To_1 : ConnectionLabel  Label=ambH_1
  CoolingPlateConnectorTop : batt_lib/Thermal/Array of Thermal Nodes Connector  numInputConnections=1  inNode1NumElements=1  inNode2NumElements=1  inNode3NumElements=1  inNode4NumElements=1  inNode5NumElements=1  inNode6NumElements=1  inNode7NumElements=1  inNode8NumElements=1  inNode9NumElements=1  inNode10NumElements=1  inNode11NumElements=1  inNode12NumElements=1  inNode13NumElements=1  inNode14NumElements=1  inNode15NumElements=1  inNode16NumElements=1  inNode17NumElements=1  inNode18NumElements=1  inNode19NumElements=1  inNode20NumElements=1  inNode21NumElements=1  inNode22NumElements=1  inNode23NumElements=1  inNode24NumElements=1  inNode25NumElements=1  inNode26NumElements=1  inNode27NumElements=1  inNode28NumElements=1  inNode29NumElements=1  inNode30NumElements=1  inNode31NumElements=1  inNode32NumElements=1  inNode33NumElements=1  inNode34NumElements=1  inNode35NumElements=1  inNode36NumElements=1  inNode37NumElements=1  inNode38NumElements=1  inNode39NumElements=1  inNode40NumElements=1  inNode41NumElements=1  inNode42NumElements=1  inNode43NumElements=1  inNode44NumElements=1  inNode45NumElements=1  inNode46NumElements=1  inNode47NumElements=1  inNode48NumElements=1  inNode49NumElements=1  inNode50NumElements=1
      settings: InternalSimscapePortConfiguration="{\"Bottom\":[{\"id\":\"outConn\",\"label\":\"outConn\",\"type\":\"foundation.thermal.thermal\"}],\"Left\":[],\"Right\":[],\"Top\":[{\"id\":\"inConn1\",\"label\":\"inConn1\",\"type\":\"foundation.thermal.thermal\"}]}"
  NewModule : Batteries_thermal_lib/Modules/ModuleType1  SOC_vecCell=[0, .1, .25, .5, .75, .9, 1]  T_vecCell=[278, 293, 313] K  V0_matCell=[3.49, 3.5, 3.51; 3.55, 3.57, 3.56; 3.62, 3.63, 3.64; 3.71, 3.71, 3.72; 3.91, 3.93, 3.94; 4.07, 4.08, 4.08; 4.19, 4.19, 4.19] V  V_rangeCell=[0, inf] V  R0_matCell=[.0117, .0085, .009; .011, .0085, .009; .0114, .0087, .0092; .0107, .0082, .0088; .0107, .0083, .0091; .0113, .0085, .0089; .0116, .0085, .0089] Ohm  AHCell=27 A*hr  extrapolation_optionCell=simscape.enum.extrapolation.nearest  thermal_massCell=100 J/K  CoolantResistance=1.2 K/W  AmbientResistance=25 K/W  P=1  S=1  iCell_specify=off  iCell_priority=None  iCell=0 A  iCell_nominal_specify=off  iCell_nominal_value=1  iCell_nominal_unit=A  vCell_specify=off  vCell_priority=None  vCell=0 V  vCell_nominal_specify=off  vCell_nominal_value=1  vCell_nominal_unit=V  socCell_specify=off  socCell_priority=High  socCell=1  socCell_nominal_specify=off  socCell_nominal_value=1  socCell_nominal_unit=1  numCyclesCell_specify=off  numCyclesCell_priority=High  numCyclesCell=0  numCyclesCell_nominal_specify=off  numCyclesCell_nominal_value=1  numCyclesCell_nominal_unit=1  temperatureCell_specify=off  temperatureCell_priority=High  temperatureCell=298.15 K  temperatureCell_nominal_specify=off  temperatureCell_nominal_value=1  temperatureCell_nominal_unit=K  vParallelAssembly_specify=off  vParallelAssembly_priority=None  vParallelAssembly=0 V  vParallelAssembly_nominal_specify=off  vParallelAssembly_nominal_value=1  vParallelAssembly_nominal_unit=V  socParallelAssembly_specify=off  socParallelAssembly_priority=None  socParallelAssembly=1  socParallelAssembly_nominal_specify=off  socParallelAssembly_nominal_value=1  socParallelAssembly_nominal_unit=1
      settings: InternalSimscapePortConfiguration="{\"Bottom\":[{\"id\":\"n\",\"label\":\"-\",\"type\":\"foundation.electrical.electrical\"}],\"Left\":[{\"id\":\"AmbH\",\"label\":\"AmbH\",\"type\":\"foundation.thermal.thermal\"}],\"Right\":[],\"Top\":[{\"id\":\"p\",\"label\":\"+\",\"type\":\"foundation.electrical.electrical\"},{\"id\":\"TopExtClnt\",\"label\":\"CPT\",\"type\":\"foundation.thermal.thermal\"}]}"
  NewModule_outputs : SimscapeProbe  BoundBlock=111  Variables={iCell, numCyclesCell, socCell, socParallelAssembly, temperatureCell, vCell, vParallelAssembly}
  iCellMux : Mux  Inputs=1
  numCyclesCellMux : Mux  Inputs=1
  socCellMux : Mux  Inputs=1
  socParallelAssemblyMux : Mux  Inputs=1
  temperatureCellMux : Mux  Inputs=1
  vCellMux : Mux  Inputs=1
  vParallelAssemblyMux : Mux  Inputs=1
  + : PMIOPort  Side=Left
  CPT : PMIOPort  Port=2  Side=Left  ConnectionType=Connection: foundation.thermal.thermal
  - : PMIOPort  Port=3  Side=Right
  AmbH : PMIOPort  Port=4  Side=Right  ConnectionType=Connection: foundation.thermal.thermal
  iCell : Outport
  numCyclesCell : Outport  Port=2
  socCell : Outport  Port=3
  socParallelAssembly : Outport  Port=4
  temperatureCell : Outport  Port=5
  vCell : Outport  Port=6
  vParallelAssembly : Outport  Port=7
  wires:
  [vParallelAssembly1] -> vParallelAssemblyMux/1
  vParallelAssemblyMux/1 -> vParallelAssembly/1
  NewModule_outputs/7 -> [vParallelAssembly1]
  [vCell1] -> vCellMux/1
  vCellMux/1 -> vCell/1
  NewModule_outputs/6 -> [vCell1]
  [temperatureCell1] -> temperatureCellMux/1
  temperatureCellMux/1 -> temperatureCell/1
  NewModule_outputs/5 -> [temperatureCell1]
  [socParallelAssembly1] -> socParallelAssemblyMux/1
  socParallelAssemblyMux/1 -> socParallelAssembly/1
  NewModule_outputs/4 -> [socParallelAssembly1]
  [socCell1] -> socCellMux/1
  socCellMux/1 -> socCell/1
  NewModule_outputs/3 -> [socCell1]
  [numCyclesCell1] -> numCyclesCellMux/1
  numCyclesCellMux/1 -> numCyclesCell/1
  NewModule_outputs/2 -> [numCyclesCell1]
  [iCell1] -> iCellMux/1
  iCellMux/1 -> iCell/1
  NewModule_outputs/1 -> [iCell1]
  connections:
  CoolingPlateConnectorTop/RConn1 -- CPT/RConn1
  CoolingPlateConnectorTop/LConn1 -- NewModule/LConn3
  AmbH_From_1/LConn1 -- AmbH/RConn1
  AmbH_To_1/LConn1 -- NewModule/LConn1
  NewModule/RConn1 -- -/RConn1
  NewModule/LConn2 -- +/RConn1
